simulink model "modelado_agitador"  (R2025b)
settings: Solver=ode4  StartTime=0.0  StopTime=10  FixedStep=1/f_t  RelTol=1e-3
PostLoadFcn:
  | parametros_modelo
InitFcn:
  | parametros_modelo
undefined symbols (not defined in the file): b_1, b_2, b_fl, c_fl, dt_c, f_t, J1, J2, k_e, k_t, Ki, Kp, L, M_zc, n_0, n_ciego, Na, P_max, P_min, P_valid_max, P_valid_min, pares_polos, R, rad, s, T_C1, T_C2, T_max, tau_stall, V_dc, w_0f, zc_tol
libraries: aerolibconvert2 x1, cstblocks x1, simulink_extras x1, eeStairGenerator x1
settings Model: Creator=Francisco  LastModifiedBy=Francisco

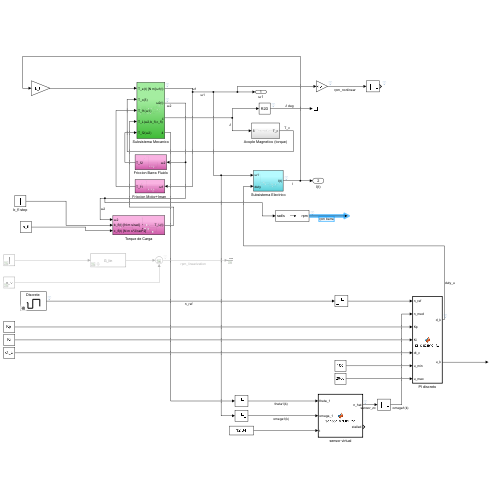
[thumbnail: Simulink's stored preview of the top-level diagram]
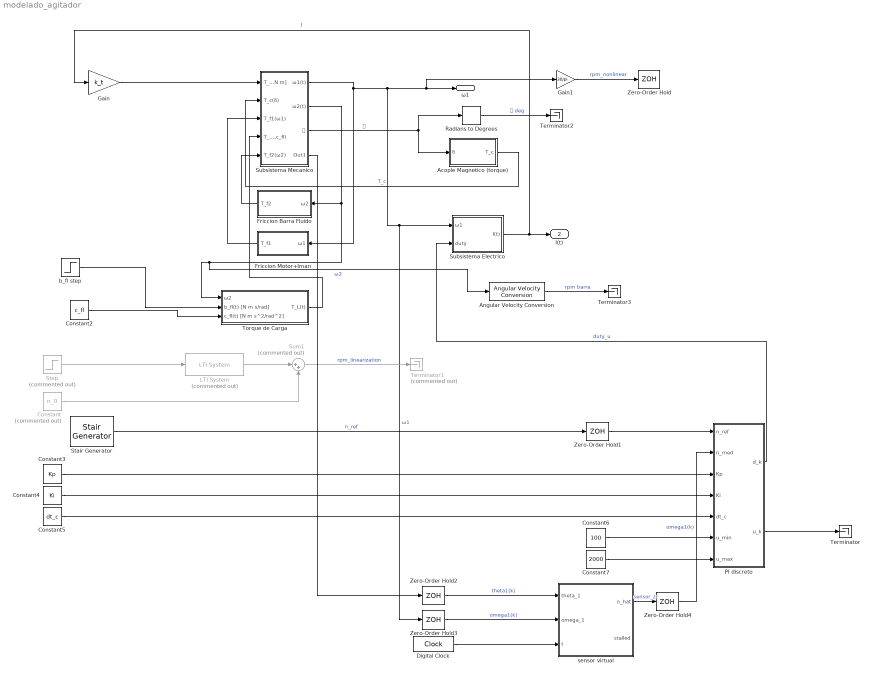
== system modelado_agitador ==
  Acople Magnetico (torque) : Subsystem
  Angular Velocity Conversion : aerolibconvert2/Angular Velocity Conversion  IU=rad/s  OU=rpm
  Constant : Constant  Commented=on  Value=n_0
  Constant2 : Constant  Value=c_fl
  Constant3 : Constant  Value=Kp
  Constant4 : Constant  Value=Ki
  Constant5 : Constant  Value=dt_c
  Constant6 : Constant  Value=100
  Constant7 : Constant  Value=2000
  Digital Clock : DigitalClock  SampleTime=1/f_t
  Friccion Barra Fluido : Subsystem
  "Friccion Motor+Iman " : Subsystem
  Gain : Gain  Gain=k_t
  Gain1 : Gain  Gain=30/pi
  LTI System : cstblocks/LTI System  Commented=on  sys=G_lin  IC=[]  PadeOrder=0
  PI discreto : MATLAB Function  TreatAsAtomicUnit=on
  Radians to Degrees : simulink_extras/Transformations/Radians to Degrees
  Stair Generator : eeStairGenerator/Stair Generator  LabelModeActiveChoice=Discrete  TimeInput=[0.5 1 3 6]  AmplitudeInput=[800 500 1000 600 ]  SampleTime=1/f_t  RepeatPattern=off  OutDataTypeStr=double
      settings: LibrarySourceBlock=ee_sl_lib/General Control/Stair Generator
  Step : Step  Commented=on  Time=4  After=0.06  SampleTime=0
  Subsistema Electrico : Subsystem
  Subsistema Mecanico : Subsystem
  Sum1 : Sum  Commented=on  Inputs=|++
  Terminator : Terminator
  Terminator1 : Terminator  Commented=on
  Terminator2 : Terminator
  Terminator3 : Terminator
  Torque de Carga : Subsystem
  Zero-Order Hold : ZeroOrderHold  SampleTime=-1
  Zero-Order Hold1 : ZeroOrderHold  SampleTime=dt_c
  Zero-Order Hold2 : ZeroOrderHold  SampleTime=1/f_t
  Zero-Order Hold3 : ZeroOrderHold  SampleTime=1/f_t
  Zero-Order Hold4 : ZeroOrderHold  SampleTime=dt_c
  b_fl step : Step  Time=4  Before=b_fl  After=b_fl  SampleTime=0
  sensor virtual : MATLAB Function  TreatAsAtomicUnit=on
  ω1 : Outport
  I(t) : Outport  Port=2
  wires:
  Gain/1 -> Subsistema Mecanico/1(T_e(t) [N m])
  Acople Magnetico (torque)/1(T_c) -> Subsistema Mecanico/2(T_c(δ))  "T_c"
  Subsistema Mecanico/1(ω1(t)) -> Zero-Order Hold3/1, Subsistema Electrico/1(ω1), Gain1/1, ω1/1, "Friccion Motor+Iman "/1(ω1)  "ω1"
  Subsistema Mecanico/3(𝛿) -> Acople Magnetico (torque)/1(δ), Radians to Degrees/1  "𝛿"
  Subsistema Mecanico/2(ω2(t)) -> Friccion Barra Fluido/1(ω2), Angular Velocity Conversion/1, Torque de Carga/1(ω2)  "ω2"
  Friccion Barra Fluido/1(T_f2) -> Subsistema Mecanico/5(T_f2(ω2))
  "Friccion Motor+Iman "/1(T_f1) -> Subsistema Mecanico/3(T_f1(ω1))
  b_fl step/1 -> Torque de Carga/2(b_fl(t) [N m s/rad])
  Constant2/1 -> Torque de Carga/3(c_fl(t) [N m s^2/rad^2])
  Torque de Carga/1(T_L(t)) -> Subsistema Mecanico/4(T_L(ω2,b_fl,c_fl))
  Subsistema Electrico/1(I(t)) -> Gain/1, I(t)/1  "I"
  Step/1 -> LTI System/1
  LTI System/1 -> Sum1/1
  Constant/1 -> Sum1/2
  Sum1/1 -> Terminator1/1  "rpm_linearization"
  Gain1/1 -> Zero-Order Hold/1  "rpm_nonlinear"
  Zero-Order Hold1/1 -> PI discreto/1(n_ref)
  PI discreto/2(u_k) -> Terminator/1
  PI discreto/1(d_k) -> Subsistema Electrico/2(duty)  "duty_u"
  Constant3/1 -> PI discreto/3(Kp)
  Constant4/1 -> PI discreto/4(Ki)
  Constant5/1 -> PI discreto/5(dt_c)
  Constant7/1 -> PI discreto/7(u_max)
  Constant6/1 -> PI discreto/6(u_min)
  Radians to Degrees/1 -> Terminator2/1  "𝛿 deg"
  Stair Generator/1 -> Zero-Order Hold1/1  "n_ref"
  Subsistema Mecanico/4(Out1) -> Zero-Order Hold2/1
  Zero-Order Hold2/1 -> sensor virtual/1(theta_1)  "theta1(k)"
  Zero-Order Hold3/1 -> sensor virtual/2(omega_1)  "omega1(k)"
  Digital Clock/1 -> sensor virtual/3(t)
  sensor virtual/1(n_hat) -> Zero-Order Hold4/1  "sensor_zc"
  Zero-Order Hold4/1 -> PI discreto/2(n_med)  "omega1(k)"
  Angular Velocity Conversion/1 -> Terminator3/1  "rpm barra"

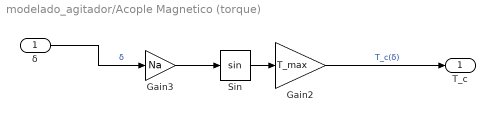
== system modelado_agitador/Acople Magnetico (torque) ==
  δ : Inport
  Gain2 : Gain  Gain=T_max
  Gain3 : Gain  Gain=Na
  Sin : Trigonometry
  T_c : Outport
  wires:
  Gain2/1 -> T_c/1  "T_c(δ)"
  Gain3/1 -> Sin/1
  Sin/1 -> Gain2/1
  δ/1 -> Gain3/1  "δ"

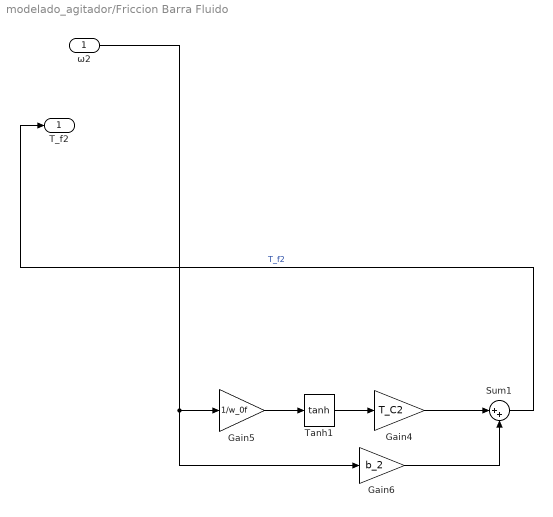
== system modelado_agitador/Friccion Barra Fluido ==
  ω2 : Inport
  Gain4 : Gain  Gain=T_C2
  Gain5 : Gain  Gain=1/w_0f
  Gain6 : Gain  Gain=b_2
  Sum1 : Sum  Inputs=|++
  Tanh1 : Trigonometry  Operator=tanh
  T_f2 : Outport
  wires:
  Gain5/1 -> Tanh1/1
  Gain4/1 -> Sum1/1
  Tanh1/1 -> Gain4/1
  Gain6/1 -> Sum1/2
  ω2/1 -> Gain6/1, Gain5/1
  Sum1/1 -> T_f2/1  "T_f2"

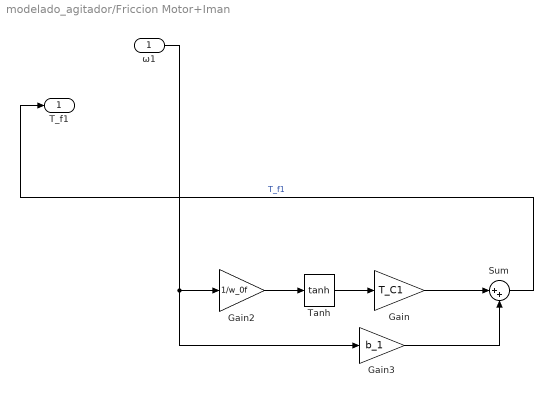
== system modelado_agitador/Friccion Motor+Iman  ==
  ω1 : Inport
  Gain : Gain  Gain=T_C1
  Gain2 : Gain  Gain=1/w_0f
  Gain3 : Gain  Gain=b_1
  Sum : Sum  Inputs=|++
  Tanh : Trigonometry  Operator=tanh
  T_f1 : Outport
  wires:
  Gain2/1 -> Tanh/1
  Gain/1 -> Sum/1
  Tanh/1 -> Gain/1
  Gain3/1 -> Sum/2
  ω1/1 -> Gain3/1, Gain2/1
  Sum/1 -> T_f1/1  "T_f1"

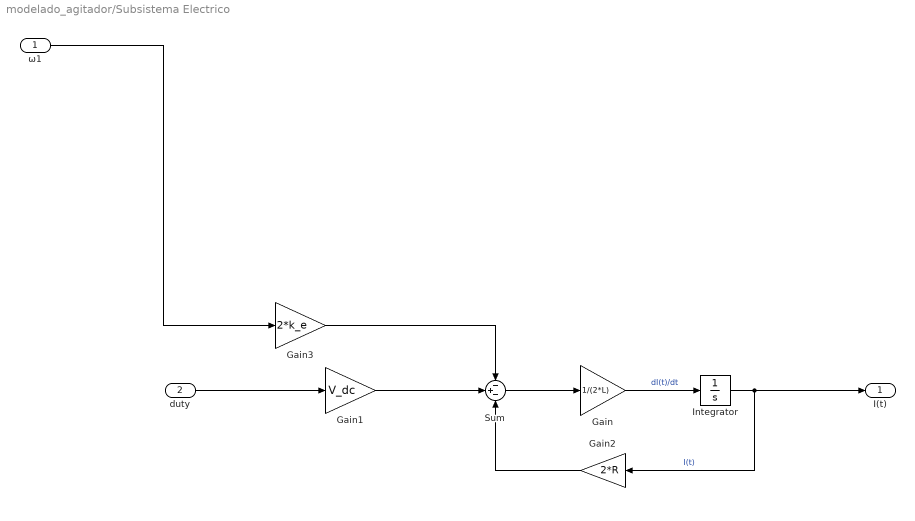
== system modelado_agitador/Subsistema Electrico ==
  ω1 : Inport
  duty : Inport  Port=2
  Gain : Gain  Gain=1/(2*L)
  Gain1 : Gain  Gain=V_dc
  Gain2 : Gain  Gain=2*R
  Gain3 : Gain  Gain=2*k_e
  Integrator : Integrator
  Sum : Sum  Inputs=-+-
  I(t) : Outport
  wires:
  Sum/1 -> Gain/1
  Gain1/1 -> Sum/2
  duty/1 -> Gain1/1
  Integrator/1 -> I(t)/1, Gain2/1  "I(t)"
  Gain/1 -> Integrator/1  "dI(t)/dt"
  Gain2/1 -> Sum/3
  Gain3/1 -> Sum/1
  ω1/1 -> Gain3/1

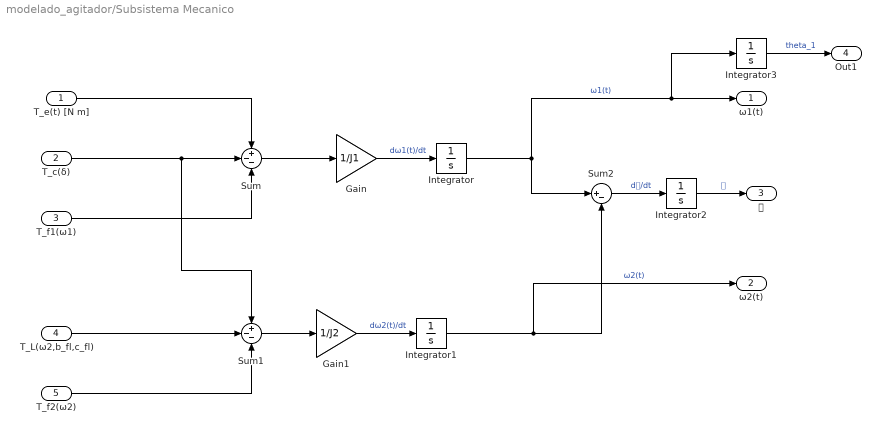
== system modelado_agitador/Subsistema Mecanico ==
  T_e(t) [N m] : Inport
  T_c(δ) : Inport  Port=2
  T_f1(ω1) : Inport  Port=3
  T_L(ω2,b_fl,c_fl) : Inport  Port=4
  T_f2(ω2) : Inport  Port=5
  Gain : Gain  Gain=1/J1
  Gain1 : Gain  Gain=1/J2
  Integrator{,1..3} (4 alike) : Integrator
  Sum : Sum  Inputs=+--
  Sum1 : Sum  Inputs=+--
  Sum2 : Sum  Inputs=|+-
  ω1(t) : Outport
  ω2(t) : Outport  Port=2
  𝛿 : Outport  Port=3
  Out1 : Outport  Port=4
  wires:
  T_c(δ)/1 -> Sum1/1, Sum/2
  T_f1(ω1)/1 -> Sum/3
  Sum/1 -> Gain/1
  T_e(t) [N m]/1 -> Sum/1
  Integrator/1 -> Sum2/1, Integrator3/1, ω1(t)/1  "ω1(t)"
  Gain/1 -> Integrator/1  "dω1(t)/dt"
  Gain1/1 -> Integrator1/1  "dω2(t)/dt"
  Integrator1/1 -> Sum2/2, ω2(t)/1  "ω2(t)"
  Sum1/1 -> Gain1/1
  T_L(ω2,b_fl,c_fl)/1 -> Sum1/2
  T_f2(ω2)/1 -> Sum1/3
  Integrator2/1 -> 𝛿/1  "𝛿"
  Sum2/1 -> Integrator2/1  "d𝛿/dt"
  Integrator3/1 -> Out1/1  "theta_1"

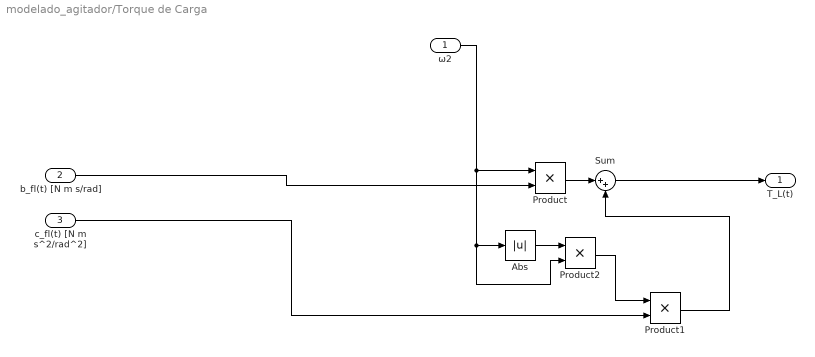
== system modelado_agitador/Torque de Carga ==
  ω2 : Inport
  b_fl(t) [N m s/rad] : Inport  Port=2
  c_fl(t) [N m s^2/rad^2] : Inport  Port=3
  Abs : Abs  SaturateOnIntegerOverflow=off
  Product : Product
  Product1 : Product
  Product2 : Product
  Sum : Sum  Inputs=|++
  T_L(t) : Outport
  wires:
  Product/1 -> Sum/1
  Product2/1 -> Product1/1
  Abs/1 -> Product2/1
  c_fl(t) [N m s^2/rad^2]/1 -> Product1/2
  b_fl(t) [N m s/rad]/1 -> Product/2
  Product1/1 -> Sum/2
  ω2/1 -> Product/1, Abs/1, Product2/2
  Sum/1 -> T_L(t)/1

== matlab function modelado_agitador/sensor virtual ==
  data: theta_1 input; n_hat output; omega_1 input; t input; stalled output; pares_polos parameter; f_t parameter; P_valid_max parameter; P_valid_min parameter; tau_stall parameter; n_ciego parameter; M_zc parameter; P_min parameter; P_max parameter; zc_tol parameter
function [n_hat, stalled] = sensor_virtual_zc(theta_1, omega_1, t, pares_polos, f_t, P_valid_max, P_valid_min, tau_stall, n_ciego, M_zc, P_min, P_max, zc_tol)
persistent last_k last_stamp periods idx count n_out last_valid_t
if isempty(last_k)
    last_k = zeros(3,1);
    last_stamp = -ones(3,1);
    periods = zeros(3, M_zc);
    idx = ones(3,1);
    count = zeros(3,1);
    n_out = 0;
    last_valid_t = 0;
end

n_real = abs(omega_1) * 30 / pi;
theta_e = pares_polos * theta_1;
phi = [0, 2*pi/3, -2*pi/3];

if n_real < n_ciego
    % Zona ciega: actualiza posicion de cruce sin capturar y resetea historial
    for k = 1:3
        last_k(k) = floor((theta_e - phi(k)) / pi);
        last_stamp(k) = -1;
        count(k) = 0;
    end
else
    for k = 1:3
        kk = floor((theta_e - phi(k)) / pi);
        if kk == last_k(k)
            continue;
        end
        last_k(k) = kk;

        stamp = mod(round(t * f_t), 65536);
        if last_stamp(k) >= 0
            P = mod(stamp - last_stamp(k), 65536);
            if P > P_valid_min && P < P_valid_max
                periods(k, idx(k)) = P;
                idx(k) = mod(idx(k), M_zc) + 1;
                count(k) = min(count(k) + 1, M_zc);
                if count(k) == M_zc
                    Pavg = floor(mean(periods(k,:)));
                    ok = all(abs(periods(k,:) - Pavg) <= zc_tol * Pavg);
                    if ok && Pavg >= P_min && Pavg <= P_max
                        n_out = floor(30 * f_t / (pares_polos * Pavg));
                        last_valid_t = t;
                    end
                end
            end
        end
        last_stamp(k) = stamp;
    end
end

if (t - last_valid_t) > tau_stall
    n_out = 0;
    stalled = 1;
else
    stalled = 0;
end
n_hat = n_out;
end

== matlab function modelado_agitador/PI discreto ==
  data: n_ref input; d_k output; n_med input; Kp input; Ki input; dt_c input; u_min input; u_max input; u_k output
function [d_k, u_k] = pi_discreto_fw(n_ref, n_med, Kp, Ki, dt_c, u_min, u_max)
persistent I_prev e_prev

if isempty(I_prev)
    I_prev = 0;
    e_prev = 0;
end

e_k = n_ref - n_med;
P_k = Kp * e_k;
I_cand = I_prev + Ki * (dt_c/2)*(e_k + e_prev);
I_k = min(u_max - P_k, max(u_min - P_k, I_cand));

u_k = min(u_max, max(u_min, P_k + I_k));
d_k = u_k / u_max;

I_prev = I_k;
e_prev = e_k;

end
